simulink model "ASM_Traffic_new"  (R2024a)
settings: Solver=ode1  StartTime=SIM.tstart.v  StopTime=SIM.tend.v  FixedStep=SIM.StepSize.v  RelTol=1e-3
PostLoadFcn:
  | if any(exist('dsrtsu_mdlpostloadfcn', 'file') ~= 0), dsrtsu_mdlpostloadfcn('Execute', bdroot); end
  | try, asm_mdl_postloadfcn(bdroot, 'UpdateModel', 3600); catch, disp(lasterr); end,
InitFcn:
  | , if any(exist('rtifpga_mdlclblib', 'file') ~= 0), rtifpga_mdlclblib('Init', bdroot); end,
  | , if any(exist('dsmpb_private', 'file') ~= 0), dsmpb_private('dsmpb_mdlclblib', 'Init', bdroot); end,
undefined symbols (not defined in the file): _to_, a0b2, ASM_BrakeHydraulics_DemoSystems, ASM_VehicleDynamics_DemoSystems, b98103fe8ad365046cd0, BrakeCircuit, CPT, Crankshaft, DiscIntNeverNeededParam, dsmsi, FinalDriveAssembly, MDL, ModeSignals, Pos_BrakePedal_Maneuver, rad, RefSignals, s_to_rpm, SIM, SoftECU, Suspension, Tire, Transmission
libraries: ASM_Traffic_lib x135, simulink x100, ASM_Utils_lib x77, ASM_VehicleDynamics_lib x70, ASM_Environment_lib x22, dsmpblib x20, dsmsilib x15, MDLD_Utils_lib x10, ASM_BrakeHydraulics_lib x3
(part 60 of 63)

== system ASM_Traffic_new/Environment/Sensors/UserInterface/DISP_Plant/Object_Sensor_3D/Object_Sensor_3D_VisualizationData/Sensor_3_Rear_NearestPoints ==
  Sensor : Inport
  Angle_Hor_Point[deg] : Gain
  Angle_Orientation_Sensor_CoorSys_V[x;y;z][deg] : Gain
  Angle_ScopeZone_Horizontal[deg] : Gain
  Bus Selector : BusSelector  OutputSignals=Parameter.Sensor_Enable[0Off|1On],Parameter.Geometry[],Parameter.Pos_Sensor_Apex_CoorSys_V[x;y;z][m],Parameter.Angle_Orientation_Sensor_CoorSys_V[x;y;z][deg],Parameter.Length_ScopeZone[m],Parameter.Length_ScopeZone_Head[m],Parameter.Angle_ScopeZone_Horizontal[deg],Parameter.Length_BlindZone[m],Parameter.SensorIdx[],SensorOutput.Object_ID[],SensorOutput.Dist_Object[m],SensorOutput.Angle_Hor_Object[deg]
  Dist_Point[m] : Gain
  Geometry[] : Gain
  Length_BlindZone[m] : Gain
  Length_ScopeZone[m] : Gain
  Length_ScopeZone_Head[m] : Gain
  Object_ID_Point[] : Gain
  Pos_Sensor_Apex_CoorSys_V[x;y;z][m] : Gain
  SensorIdx[] : Gain
  Sensor_Enable[0Off|1On] : Gain
  Terminator{9..20} (12 alike) : Terminator
  wires:
  Sensor/1 -> Bus Selector/1
  Length_BlindZone[m]/1 -> Terminator12/1
  Angle_ScopeZone_Horizontal[deg]/1 -> Terminator15/1
  Sensor_Enable[0Off|1On]/1 -> Terminator10/1
  Length_ScopeZone[m]/1 -> Terminator17/1
  Dist_Point[m]/1 -> Terminator9/1
  Angle_Orientation_Sensor_CoorSys_V[x;y;z][deg]/1 -> Terminator18/1
  Angle_Hor_Point[deg]/1 -> Terminator19/1
  SensorIdx[]/1 -> Terminator14/1
  Length_ScopeZone_Head[m]/1 -> Terminator16/1
  Pos_Sensor_Apex_CoorSys_V[x;y;z][m]/1 -> Terminator20/1
  Geometry[]/1 -> Terminator11/1
  Object_ID_Point[]/1 -> Terminator13/1
  Bus Selector/1 -> Sensor_Enable[0Off|1On]/1  "<Sensor_Enable[0Off|1On]>"
  Bus Selector/2 -> Geometry[]/1  "<Geometry[]>"
  Bus Selector/3 -> Pos_Sensor_Apex_CoorSys_V[x;y;z][m]/1  "<Pos_Sensor_Apex_CoorSys_V[x;y;z][m]>"
  Bus Selector/4 -> Angle_Orientation_Sensor_CoorSys_V[x;y;z][deg]/1  "<Angle_Orientation_Sensor_CoorSys_V[x;y;z][deg]>"
  Bus Selector/5 -> Length_ScopeZone[m]/1  "<Length_ScopeZone[m]>"
  Bus Selector/6 -> Length_ScopeZone_Head[m]/1  "<Length_ScopeZone_Head[m]>"
  Bus Selector/7 -> Angle_ScopeZone_Horizontal[deg]/1  "<Angle_ScopeZone_Horizontal[deg]>"
  Bus Selector/8 -> Length_BlindZone[m]/1  "<Length_BlindZone[m]>"
  Bus Selector/9 -> SensorIdx[]/1  "<SensorIdx[]>"
  Bus Selector/11 -> Dist_Point[m]/1  "<Dist_Object[m]>"
  Bus Selector/10 -> Object_ID_Point[]/1  "<Object_ID[]>"
  Bus Selector/12 -> Angle_Hor_Point[deg]/1  "<Angle_Hor_Object[deg]>"

== system ASM_Traffic_new/Environment/Sensors/UserInterface/DISP_Plant/Object_Sensor_3D/Object_Sensor_3D_VisualizationData/Sensor_3_Rear_RadarReflectionPoints ==
  Sensor : Inport
  Angle_Hor_Point[deg] : Gain
  Angle_Orientation_Sensor_CoorSys_V[x;y;z][deg] : Gain
  Angle_ScopeZone_Horizontal[deg] : Gain
  Bus Selector : BusSelector  OutputSignals=Parameter.Sensor_Enable[0Off|1On],Parameter.Geometry[],Parameter.Pos_Sensor_Apex_CoorSys_V[x;y;z][m],Parameter.Angle_Orientation_Sensor_CoorSys_V[x;y;z][deg],Parameter.Length_ScopeZone[m],Parameter.Length_ScopeZone_Head[m],Parameter.Angle_ScopeZone_Horizontal[deg],Parameter.Length_BlindZone[m],Parameter.SensorIdx[],RadarEffects.Object_ID[],RadarEffects.Dist_CoorSys_S[m],RadarEffects.Angle_Hor_CoorSys_S[deg]
  Dist_Point[m] : Gain
  Geometry[] : Gain
  Length_BlindZone[m] : Gain
  Length_ScopeZone[m] : Gain
  Length_ScopeZone_Head[m] : Gain
  Object_ID_Point[] : Gain
  Pos_Sensor_Apex_CoorSys_V[x;y;z][m] : Gain
  SensorIdx[] : Gain
  Sensor_Enable[0Off|1On] : Gain
  Terminator{9..20} (12 alike) : Terminator
  wires:
  Bus Selector/12 -> Angle_Hor_Point[deg]/1  "<Angle_Hor_CoorSys_S[deg]>"
  Bus Selector/10 -> Object_ID_Point[]/1  "<Object_ID[]>"
  Bus Selector/11 -> Dist_Point[m]/1  "<Dist_CoorSys_S[m]>"
  Bus Selector/9 -> SensorIdx[]/1  "<SensorIdx[]>"
  Bus Selector/8 -> Length_BlindZone[m]/1  "<Length_BlindZone[m]>"
  Bus Selector/7 -> Angle_ScopeZone_Horizontal[deg]/1  "<Angle_ScopeZone_Horizontal[deg]>"
  Bus Selector/6 -> Length_ScopeZone_Head[m]/1  "<Length_ScopeZone_Head[m]>"
  Bus Selector/5 -> Length_ScopeZone[m]/1  "<Length_ScopeZone[m]>"
  Bus Selector/4 -> Angle_Orientation_Sensor_CoorSys_V[x;y;z][deg]/1  "<Angle_Orientation_Sensor_CoorSys_V[x;y;z][deg]>"
  Bus Selector/3 -> Pos_Sensor_Apex_CoorSys_V[x;y;z][m]/1  "<Pos_Sensor_Apex_CoorSys_V[x;y;z][m]>"
  Bus Selector/2 -> Geometry[]/1  "<Geometry[]>"
  Bus Selector/1 -> Sensor_Enable[0Off|1On]/1  "<Sensor_Enable[0Off|1On]>"
  Object_ID_Point[]/1 -> Terminator13/1
  Geometry[]/1 -> Terminator11/1
  Pos_Sensor_Apex_CoorSys_V[x;y;z][m]/1 -> Terminator20/1
  Length_ScopeZone_Head[m]/1 -> Terminator16/1
  SensorIdx[]/1 -> Terminator14/1
  Angle_Hor_Point[deg]/1 -> Terminator19/1
  Angle_Orientation_Sensor_CoorSys_V[x;y;z][deg]/1 -> Terminator18/1
  Dist_Point[m]/1 -> Terminator9/1
  Length_ScopeZone[m]/1 -> Terminator17/1
  Sensor_Enable[0Off|1On]/1 -> Terminator10/1
  Angle_ScopeZone_Horizontal[deg]/1 -> Terminator15/1
  Length_BlindZone[m]/1 -> Terminator12/1
  Sensor/1 -> Bus Selector/1

== system ASM_Traffic_new/Environment/Sensors/UserInterface/DISP_Plant/Traffic_Sign_Sensor/GetTrfSgnDataByIndex_1/SwitchObjectData ==
  TrafficBus : Inport
  Switch : Inport  Port=2
  Bus Selector2 : BusSelector  OutputSignals=TrafficSign_Sensor_Dyn.Sensor_Front_1.SensorOutput[].TrafficObject_Type[]
  Bus Selector3 : BusSelector  OutputSignals=TrafficSign_Sensor_Dyn.Sensor_Front_1.SensorOutput[].TrafficObject_ID[]
  Bus Selector4 : BusSelector  OutputSignals=TrafficSign_Sensor_Dyn.Sensor_Front_1.SensorOutput[].Parent_Object_ID[]
  Bus Selector44 : BusSelector  OutputSignals=TrafficSign_Sensor_Dyn.Sensor_Front_1.SensorOutput[].Traffic_Sign_Valid[0|1]
  Selector{,1..3} (4 alike) : Selector  InputPortWidth=MDL.Traffic.Sensors.TrafficSignSensorDyn_Calculation.Const_Sensor_Output_Dimension.v  IndexOptions=Index vector (port)  Indices=[1 3]  OutputSizes=1
  Traffic_Sign_Valid[0|1] : Outport  VectorParamsAs1DForOutWhenUnconnected=off
  TrafficObject_ID[] : Outport  Port=2  VectorParamsAs1DForOutWhenUnconnected=off
  TrafficObject_Type[] : Outport  Port=3  VectorParamsAs1DForOutWhenUnconnected=off
  Parent_Object_ID[] : Outport  Port=4  VectorParamsAs1DForOutWhenUnconnected=off
  wires:
  Selector3/1 -> Parent_Object_ID[]/1
  Bus Selector4/1 -> Selector3/1  "<Parent_Object_ID[]>"
  Selector2/1 -> TrafficObject_Type[]/1
  Switch/1 -> Selector/2, Selector1/2, Selector2/2, Selector3/2
  Selector/1 -> Traffic_Sign_Valid[0|1]/1
  Bus Selector44/1 -> Selector/1  "<Traffic_Sign_Valid[0|1]>"
  Selector1/1 -> TrafficObject_ID[]/1
  Bus Selector3/1 -> Selector1/1  "<TrafficObject_ID[]>"
  TrafficBus/1 -> Bus Selector44/1, Bus Selector3/1, Bus Selector2/1, Bus Selector4/1
  Bus Selector2/1 -> Selector2/1  "<TrafficObject_Type[]>"

== system ASM_Traffic_new/Environment/Sensors/UserInterface/DISP_Plant/Traffic_Sign_Sensor/GetTrfSgnDataByIndex_1/SwitchObjectPosition ==
  TrafficBus : Inport
  Switch : Inport  Port=2
  Bus Selector1 : BusSelector  OutputSignals=TrafficSign_Sensor_Dyn.Sensor_Front_1.SensorOutput[].Pos_CoorSys_S[x;y;z][m]
  Bus Selector2 : BusSelector  OutputSignals=TrafficSign_Sensor_Dyn.Sensor_Front_1.SensorOutput[].Angle_Hor_Rel[deg]
  Bus Selector3 : BusSelector  OutputSignals=TrafficSign_Sensor_Dyn.Sensor_Front_1.SensorOutput[].Angle_CoorSys_E[x;y;z][deg]
  Bus Selector4 : BusSelector  OutputSignals=TrafficSign_Sensor_Dyn.Sensor_Front_1.SensorOutput[].Angle_Ver_Rel[deg]
  Bus Selector44 : BusSelector  OutputSignals=TrafficSign_Sensor_Dyn.Sensor_Front_1.SensorOutput[].Pos_CoorSys_E[x;y;z][m]
  Bus Selector5 : BusSelector  OutputSignals=TrafficSign_Sensor_Dyn.Sensor_Front_1.SensorOutput[].Distance[m]
  Idx_comp : Subsystem
  Idx_comp1 : Subsystem
  Idx_comp2 : Subsystem
  Mux : Mux  Inputs=3
  Mux1 : Mux  Inputs=3
  Mux2 : Mux  Inputs=3
  Selector{1..9} (9 alike) : Selector  InputPortWidth=MDL.Traffic.Sensors.TrafficSignSensorDyn_Calculation.Const_Sensor_Output_Dimension.v*3  IndexOptions=Index vector (port)  Indices=[1 3]  OutputSizes=1
  Selector10 : Selector  InputPortWidth=MDL.Traffic.Sensors.TrafficSignSensorDyn_Calculation.Const_Sensor_Output_Dimension.v  IndexOptions=Index vector (port)  Indices=[1 3]  OutputSizes=1
  Selector11 : Selector  InputPortWidth=MDL.Traffic.Sensors.TrafficSignSensorDyn_Calculation.Const_Sensor_Output_Dimension.v  IndexOptions=Index vector (port)  Indices=[1 3]  OutputSizes=1
  Selector12 : Selector  InputPortWidth=MDL.Traffic.Sensors.TrafficSignSensorDyn_Calculation.Const_Sensor_Output_Dimension.v  IndexOptions=Index vector (port)  Indices=[1 3]  OutputSizes=1
  Pos_CoorSys_E[x;y;z][m] : Outport  VectorParamsAs1DForOutWhenUnconnected=off
  Angle_CoorSys_E[x;y;z][deg] : Outport  Port=2  VectorParamsAs1DForOutWhenUnconnected=off
  Pos_CoorSys_S[x;y;z][m] : Outport  Port=3  VectorParamsAs1DForOutWhenUnconnected=off
  Angle_Hor_Rel[deg] : Outport  Port=4  VectorParamsAs1DForOutWhenUnconnected=off
  Angle_Ver_Rel[deg] : Outport  Port=5  VectorParamsAs1DForOutWhenUnconnected=off
  Distance[m] : Outport  Port=6  VectorParamsAs1DForOutWhenUnconnected=off
  wires:
  Selector12/1 -> Distance[m]/1
  Selector11/1 -> Angle_Ver_Rel[deg]/1
  Selector10/1 -> Angle_Hor_Rel[deg]/1
  Bus Selector5/1 -> Selector12/1  "<Distance[m]>"
  Bus Selector4/1 -> Selector11/1  "<Angle_Ver_Rel[deg]>"
  Bus Selector2/1 -> Selector10/1  "<Angle_Hor_Rel[deg]>"
  Mux2/1 -> Pos_CoorSys_S[x;y;z][m]/1
  Idx_comp2/3(Idx_comp_z) -> Selector9/2
  Idx_comp2/2(Idx_comp_y) -> Selector8/2
  Idx_comp2/1(Idx_comp_x) -> Selector7/2
  Selector9/1 -> Mux2/3
  Selector8/1 -> Mux2/2
  Selector7/1 -> Mux2/1
  Bus Selector1/1 -> Selector7/1, Selector8/1, Selector9/1  "<Pos_CoorSys_S[x;y;z][m]>"
  Mux1/1 -> Angle_CoorSys_E[x;y;z][deg]/1
  Selector3/1 -> Mux1/3
  Selector2/1 -> Mux1/2
  Selector1/1 -> Mux1/1
  Idx_comp1/3(Idx_comp_z) -> Selector3/2
  Idx_comp1/2(Idx_comp_y) -> Selector2/2
  Idx_comp1/1(Idx_comp_x) -> Selector1/2
  Mux/1 -> Pos_CoorSys_E[x;y;z][m]/1
  Selector6/1 -> Mux/3
  Selector5/1 -> Mux/2
  Selector4/1 -> Mux/1
  Idx_comp/3(Idx_comp_z) -> Selector6/2
  Idx_comp/2(Idx_comp_y) -> Selector5/2
  Idx_comp/1(Idx_comp_x) -> Selector4/2
  TrafficBus/1 -> Bus Selector3/1, Bus Selector4/1, Bus Selector5/1, Bus Selector2/1, Bus Selector1/1, Bus Selector44/1
  Bus Selector3/1 -> Selector1/1, Selector2/1, Selector3/1  "<Angle_CoorSys_E[x;y;z][deg]>"
  Bus Selector44/1 -> Selector4/1, Selector5/1, Selector6/1  "<Pos_CoorSys_E[x;y;z][m]>"
  Switch/1 -> Idx_comp/1(Idx), Idx_comp1/1(Idx), Idx_comp2/1(Idx), Selector10/2, Selector11/2, Selector12/2

== system ASM_Traffic_new/Environment/Sensors/UserInterface/DISP_Plant/Traffic_Sign_Sensor/GetTrfSgnDataByIndex_1/SwitchSignProperties ==
  TrafficBus : Inport
  Switch : Inport  Port=2
  Bus Selector1 : BusSelector  OutputSignals=TrafficSign_Sensor_Dyn.Sensor_Front_1.SensorOutput[].Traffic_Sign_Visibility[0_100]
  Bus Selector2 : BusSelector  OutputSignals=TrafficSign_Sensor_Dyn.Sensor_Front_1.SensorOutput[].Traffic_Sign_Value[]
  Bus Selector3 : BusSelector  OutputSignals=TrafficSign_Sensor_Dyn.Sensor_Front_1.SensorOutput[].Traffic_Sign_Subtype[]
  Bus Selector4 : BusSelector  OutputSignals=TrafficSign_Sensor_Dyn.Sensor_Front_1.SensorOutput[].Traffic_Sign_Country[]
  Bus Selector44 : BusSelector  OutputSignals=TrafficSign_Sensor_Dyn.Sensor_Front_1.SensorOutput[].Traffic_Sign_Type[]
  Bus Selector5 : BusSelector  OutputSignals=TrafficSign_Sensor_Dyn.Sensor_Front_1.SensorOutput[].Traffic_Sign_Lanes[]
  Bus Selector6 : BusSelector  OutputSignals=TrafficSign_Sensor_Dyn.Sensor_Front_1.SensorOutput[].Object_State[]
  Bus Selector7 : BusSelector  OutputSignals=TrafficSign_Sensor_Dyn.Sensor_Front_1.SensorOutput[].Object_Stream_ID[]
  Idx_comp : Subsystem
  Mux2 : Mux  Inputs=5
  Selector{,1..3,6,10..11} (7 alike) : Selector  InputPortWidth=MDL.Traffic.Sensors.TrafficSignSensorDyn_Calculation.Const_Sensor_Output_Dimension.v  IndexOptions=Index vector (port)  Indices=[1 3]  OutputSizes=1
  Selector{4..5,7..9} (5 alike) : Selector  InputPortWidth=MDL.Traffic.Sensors.TrafficSignSensorDyn_Calculation.Const_Sensor_Output_Dimension.v*5  IndexOptions=Index vector (port)  Indices=[1 3]  OutputSizes=1
  Traffic_Sign_Type[] : Outport  VectorParamsAs1DForOutWhenUnconnected=off
  Traffic_Sign_Subtype[] : Outport  Port=2  VectorParamsAs1DForOutWhenUnconnected=off
  Traffic_Sign_Value[] : Outport  Port=3  VectorParamsAs1DForOutWhenUnconnected=off
  Traffic_Sign_Country[] : Outport  Port=4  VectorParamsAs1DForOutWhenUnconnected=off
  Traffic_Sign_Visibility[0_100] : Outport  Port=5  VectorParamsAs1DForOutWhenUnconnected=off
  Object_State[] : Outport  Port=6  VectorParamsAs1DForOutWhenUnconnected=off
  Object_Stream_ID[] : Outport  Port=7  VectorParamsAs1DForOutWhenUnconnected=off
  Traffic_Sign_Lanes[] : Outport  Port=8  VectorParamsAs1DForOutWhenUnconnected=off
  wires:
  Bus Selector7/1 -> Selector11/1  "<Object_Stream_ID[]>"
  Selector11/1 -> Object_Stream_ID[]/1
  Bus Selector6/1 -> Selector10/1  "<Object_State[]>"
  Selector10/1 -> Object_State[]/1
  Selector6/1 -> Traffic_Sign_Visibility[0_100]/1
  Selector4/1 -> Mux2/4
  Idx_comp/4(Idx_comp_4) -> Selector4/2
  Idx_comp/5(Idx_comp_5) -> Selector5/2
  Selector5/1 -> Mux2/5
  Mux2/1 -> Traffic_Sign_Lanes[]/1
  Idx_comp/3(Idx_comp_3) -> Selector9/2
  Idx_comp/2(Idx_comp_2) -> Selector8/2
  Idx_comp/1(Idx_comp_1) -> Selector7/2
  Selector9/1 -> Mux2/3
  Selector8/1 -> Mux2/2
  Selector7/1 -> Mux2/1
  Bus Selector5/1 -> Selector7/1, Selector8/1, Selector9/1, Selector5/1, Selector4/1  "<Traffic_Sign_Lanes[]>"
  Bus Selector1/1 -> Selector6/1  "<Traffic_Sign_Visibility[0_100]>"
  Bus Selector2/1 -> Selector2/1  "<Traffic_Sign_Value[]>"
  TrafficBus/1 -> Bus Selector4/1, Bus Selector1/1, Bus Selector7/1, Bus Selector5/1, Bus Selector6/1, Bus Selector2/1, Bus Selector3/1, Bus Selector44/1
  Bus Selector3/1 -> Selector1/1  "<Traffic_Sign_Subtype[]>"
  Selector1/1 -> Traffic_Sign_Subtype[]/1
  Bus Selector44/1 -> Selector/1  "<Traffic_Sign_Type[]>"
  Selector/1 -> Traffic_Sign_Type[]/1
  Switch/1 -> Selector3/2, Selector10/2, Idx_comp/1(Idx), Selector11/2, Selector6/2, Selector2/2, Selector1/2, Selector/2
  Selector2/1 -> Traffic_Sign_Value[]/1
  Bus Selector4/1 -> Selector3/1  "<Traffic_Sign_Country[]>"
  Selector3/1 -> Traffic_Sign_Country[]/1

== system ASM_Traffic_new/Environment/Traffic/UserInterface/DISP_Plant/Fellow_Movement/GetFellowDataByIndex_1/SwitchFellowMovementData ==
  TrafficBus : Inport
  Switch : Inport  Port=2
  Bus Selector2 : BusSelector  OutputSignals=Traffic_Signals_toEnvironment.Flag_FellowUsed[0|1]
  Bus Selector3 : BusSelector  OutputSignals=FellowSignalLabels.s_Fellows[m]
  Bus Selector4 : BusSelector  OutputSignals=FellowSignalLabels.d_Total_Fellows[m]
  Bus Selector5 : BusSelector  OutputSignals=FellowSignalLabels.v_Fellows[km|h]
  Flag_Fellow_Used[0|1] : Subsystem
      mask Display: disp('')
  Selector{,1..3} (4 alike) : Selector  InputPortWidth=MDL.Traffic.MaxNumFellows.v  IndexOptions=Index vector (port)  Indices=[1 3]  OutputSizes=1
  d_Total_Fellow[m] : Subsystem
      mask Display: disp('')
  s_Fellow[m] : Subsystem
      mask Display: disp('')
  v_Fellow[km|h] : Subsystem
      mask Display: disp('')
  "Flag_Fellow_Used[0|1] " : Outport  VectorParamsAs1DForOutWhenUnconnected=off
  "s_Fellow[m] " : Outport  Port=2  VectorParamsAs1DForOutWhenUnconnected=off
  "d_Total_Fellow[m] " : Outport  Port=3  VectorParamsAs1DForOutWhenUnconnected=off
  "v_Fellow[km|h] " : Outport  Port=4  VectorParamsAs1DForOutWhenUnconnected=off
  wires:
  TrafficBus/1 -> Bus Selector2/1, Bus Selector3/1, Bus Selector4/1, Bus Selector5/1
  Selector3/1 -> v_Fellow[km|h]/1(In1)
  Bus Selector5/1 -> Selector3/1  "<v_Fellows[km|h]>"
  Selector2/1 -> d_Total_Fellow[m]/1(In1)
  Bus Selector4/1 -> Selector2/1  "<d_Total_Fellows[m]>"
  Selector1/1 -> s_Fellow[m]/1(In1)
  Bus Selector3/1 -> Selector1/1  "<s_Fellows[m]>"
  Selector/1 -> Flag_Fellow_Used[0|1]/1(In1)
  Bus Selector2/1 -> Selector/1  "<Flag_FellowUsed[0|1]>"
  Switch/1 -> Selector/2, Selector1/2, Selector2/2, Selector3/2
  v_Fellow[km|h]/1(Out1) -> "v_Fellow[km|h] "/1  "v_Fellow[km|h]"
  d_Total_Fellow[m]/1(Out1) -> "d_Total_Fellow[m] "/1  "d_Total_Fellow[m]"
  s_Fellow[m]/1(Out1) -> "s_Fellow[m] "/1  "s_Fellow[m]"
  Flag_Fellow_Used[0|1]/1(Out1) -> "Flag_Fellow_Used[0|1] "/1  "Flag_Fellow_Used[0|1]"

== system ASM_Traffic_new/Environment/Traffic/UserInterface/DISP_Plant/Fellow_Movement/GetFellowDataByIndex_1/SwitchInfoData ==
  TrafficBus : Inport
  Switch : Inport  Port=2
  Bus Selector1 : BusSelector  OutputSignals=Traffic_Signals_toEnvironment.Info.CurrentSegment_Fellows[]
  Bus Selector2 : BusSelector  OutputSignals=Traffic_Signals_toEnvironment.Info.t_local_Fellows[s]
  Bus Selector44 : BusSelector  OutputSignals=Traffic_Signals_toEnvironment.Info.CurrentSequence_Fellows[]
  Selector : Selector  InputPortWidth=MDL.Traffic.MaxNumFellows.v  IndexOptions=Index vector (port)  Indices=[1 3]  OutputSizes=1
  Selector1 : Selector  InputPortWidth=MDL.Traffic.MaxNumFellows.v  IndexOptions=Index vector (port)  Indices=[1 3]  OutputSizes=1
  Selector2 : Selector  InputPortWidth=MDL.Traffic.MaxNumFellows.v  IndexOptions=Index vector (port)  Indices=[1 3]  OutputSizes=1
  CurrentSequence[] : Outport  VectorParamsAs1DForOutWhenUnconnected=off
  CurrentSegment[] : Outport  Port=2  VectorParamsAs1DForOutWhenUnconnected=off
  t_local[s] : Outport  Port=3  VectorParamsAs1DForOutWhenUnconnected=off
  wires:
  Selector2/1 -> t_local[s]/1
  Switch/1 -> Selector/2, Selector1/2, Selector2/2
  Selector/1 -> CurrentSequence[]/1
  Bus Selector44/1 -> Selector/1  "<CurrentSequence_Fellows[]>"
  Selector1/1 -> CurrentSegment[]/1
  Bus Selector1/1 -> Selector1/1  "<CurrentSegment_Fellows[]>"
  TrafficBus/1 -> Bus Selector44/1, Bus Selector1/1, Bus Selector2/1
  Bus Selector2/1 -> Selector2/1  "<t_local_Fellows[s]>"

== system ASM_Traffic_new/Environment/Traffic/UserInterface/DISP_Plant/Fellow_Movement/GetFellowDataByIndex_2/SwitchFellowMovementData ==
  TrafficBus : Inport
  Switch : Inport  Port=2
  Bus Selector2 : BusSelector  OutputSignals=Traffic_Signals_toEnvironment.Flag_FellowUsed[0|1]
  Bus Selector3 : BusSelector  OutputSignals=FellowSignalLabels.s_Fellows[m]
  Bus Selector4 : BusSelector  OutputSignals=FellowSignalLabels.d_Total_Fellows[m]
  Bus Selector5 : BusSelector  OutputSignals=FellowSignalLabels.v_Fellows[km|h]
  Flag_Fellow_Used[0|1] : Subsystem
      mask Display: disp('')
  Selector{,1..3} (4 alike) : Selector  InputPortWidth=MDL.Traffic.MaxNumFellows.v  IndexOptions=Index vector (port)  Indices=[1 3]  OutputSizes=1
  d_Total_Fellow[m] : Subsystem
      mask Display: disp('')
  s_Fellow[m] : Subsystem
      mask Display: disp('')
  v_Fellow[km|h] : Subsystem
      mask Display: disp('')
  "Flag_Fellow_Used[0|1] " : Outport  VectorParamsAs1DForOutWhenUnconnected=off
  "s_Fellow[m] " : Outport  Port=2  VectorParamsAs1DForOutWhenUnconnected=off
  "d_Total_Fellow[m] " : Outport  Port=3  VectorParamsAs1DForOutWhenUnconnected=off
  "v_Fellow[km|h] " : Outport  Port=4  VectorParamsAs1DForOutWhenUnconnected=off
  wires:
  TrafficBus/1 -> Bus Selector2/1, Bus Selector3/1, Bus Selector4/1, Bus Selector5/1
  Selector3/1 -> v_Fellow[km|h]/1(In1)
  Bus Selector5/1 -> Selector3/1  "<v_Fellows[km|h]>"
  Selector2/1 -> d_Total_Fellow[m]/1(In1)
  Bus Selector4/1 -> Selector2/1  "<d_Total_Fellows[m]>"
  Selector1/1 -> s_Fellow[m]/1(In1)
  Bus Selector3/1 -> Selector1/1  "<s_Fellows[m]>"
  Selector/1 -> Flag_Fellow_Used[0|1]/1(In1)
  Bus Selector2/1 -> Selector/1  "<Flag_FellowUsed[0|1]>"
  Switch/1 -> Selector/2, Selector1/2, Selector2/2, Selector3/2
  v_Fellow[km|h]/1(Out1) -> "v_Fellow[km|h] "/1  "v_Fellow[km|h]"
  d_Total_Fellow[m]/1(Out1) -> "d_Total_Fellow[m] "/1  "d_Total_Fellow[m]"
  s_Fellow[m]/1(Out1) -> "s_Fellow[m] "/1  "s_Fellow[m]"
  Flag_Fellow_Used[0|1]/1(Out1) -> "Flag_Fellow_Used[0|1] "/1  "Flag_Fellow_Used[0|1]"

== system ASM_Traffic_new/Environment/Traffic/UserInterface/DISP_Plant/Fellow_Movement/GetFellowDataByIndex_2/SwitchInfoData ==
  TrafficBus : Inport
  Switch : Inport  Port=2
  Bus Selector1 : BusSelector  OutputSignals=Traffic_Signals_toEnvironment.Info.CurrentSegment_Fellows[]
  Bus Selector2 : BusSelector  OutputSignals=Traffic_Signals_toEnvironment.Info.t_local_Fellows[s]
  Bus Selector44 : BusSelector  OutputSignals=Traffic_Signals_toEnvironment.Info.CurrentSequence_Fellows[]
  Selector : Selector  InputPortWidth=MDL.Traffic.MaxNumFellows.v  IndexOptions=Index vector (port)  Indices=[1 3]  OutputSizes=1
  Selector1 : Selector  InputPortWidth=MDL.Traffic.MaxNumFellows.v  IndexOptions=Index vector (port)  Indices=[1 3]  OutputSizes=1
  Selector2 : Selector  InputPortWidth=MDL.Traffic.MaxNumFellows.v  IndexOptions=Index vector (port)  Indices=[1 3]  OutputSizes=1
  CurrentSequence[] : Outport  VectorParamsAs1DForOutWhenUnconnected=off
  CurrentSegment[] : Outport  Port=2  VectorParamsAs1DForOutWhenUnconnected=off
  t_local[s] : Outport  Port=3  VectorParamsAs1DForOutWhenUnconnected=off
  wires:
  Selector2/1 -> t_local[s]/1
  Switch/1 -> Selector/2, Selector1/2, Selector2/2
  Selector/1 -> CurrentSequence[]/1
  Bus Selector44/1 -> Selector/1  "<CurrentSequence_Fellows[]>"
  Selector1/1 -> CurrentSegment[]/1
  Bus Selector1/1 -> Selector1/1  "<CurrentSegment_Fellows[]>"
  TrafficBus/1 -> Bus Selector44/1, Bus Selector1/1, Bus Selector2/1
  Bus Selector2/1 -> Selector2/1  "<t_local_Fellows[s]>"

== system ASM_Traffic_new/Environment/Traffic/UserInterface/DISP_Plant/Fellow_Movement/GetFellowDataByIndex_3/SwitchFellowMovementData ==
  TrafficBus : Inport
  Switch : Inport  Port=2
  Bus Selector2 : BusSelector  OutputSignals=Traffic_Signals_toEnvironment.Flag_FellowUsed[0|1]
  Bus Selector3 : BusSelector  OutputSignals=FellowSignalLabels.s_Fellows[m]
  Bus Selector4 : BusSelector  OutputSignals=FellowSignalLabels.d_Total_Fellows[m]
  Bus Selector5 : BusSelector  OutputSignals=FellowSignalLabels.v_Fellows[km|h]
  Flag_Fellow_Used[0|1] : Subsystem
      mask Display: disp('')
  Selector{,1..3} (4 alike) : Selector  InputPortWidth=MDL.Traffic.MaxNumFellows.v  IndexOptions=Index vector (port)  Indices=[1 3]  OutputSizes=1
  d_Total_Fellow[m] : Subsystem
      mask Display: disp('')
  s_Fellow[m] : Subsystem
      mask Display: disp('')
  v_Fellow[km|h] : Subsystem
      mask Display: disp('')
  "Flag_Fellow_Used[0|1] " : Outport  VectorParamsAs1DForOutWhenUnconnected=off
  "s_Fellow[m] " : Outport  Port=2  VectorParamsAs1DForOutWhenUnconnected=off
  "d_Total_Fellow[m] " : Outport  Port=3  VectorParamsAs1DForOutWhenUnconnected=off
  "v_Fellow[km|h] " : Outport  Port=4  VectorParamsAs1DForOutWhenUnconnected=off
  wires:
  TrafficBus/1 -> Bus Selector2/1, Bus Selector3/1, Bus Selector4/1, Bus Selector5/1
  Selector3/1 -> v_Fellow[km|h]/1(In1)
  Bus Selector5/1 -> Selector3/1  "<v_Fellows[km|h]>"
  Selector2/1 -> d_Total_Fellow[m]/1(In1)
  Bus Selector4/1 -> Selector2/1  "<d_Total_Fellows[m]>"
  Selector1/1 -> s_Fellow[m]/1(In1)
  Bus Selector3/1 -> Selector1/1  "<s_Fellows[m]>"
  Selector/1 -> Flag_Fellow_Used[0|1]/1(In1)
  Bus Selector2/1 -> Selector/1  "<Flag_FellowUsed[0|1]>"
  Switch/1 -> Selector/2, Selector1/2, Selector2/2, Selector3/2
  v_Fellow[km|h]/1(Out1) -> "v_Fellow[km|h] "/1  "v_Fellow[km|h]"
  d_Total_Fellow[m]/1(Out1) -> "d_Total_Fellow[m] "/1  "d_Total_Fellow[m]"
  s_Fellow[m]/1(Out1) -> "s_Fellow[m] "/1  "s_Fellow[m]"
  Flag_Fellow_Used[0|1]/1(Out1) -> "Flag_Fellow_Used[0|1] "/1  "Flag_Fellow_Used[0|1]"

== system ASM_Traffic_new/Environment/Traffic/UserInterface/DISP_Plant/Fellow_Movement/GetFellowDataByIndex_3/SwitchInfoData ==
  TrafficBus : Inport
  Switch : Inport  Port=2
  Bus Selector1 : BusSelector  OutputSignals=Traffic_Signals_toEnvironment.Info.CurrentSegment_Fellows[]
  Bus Selector2 : BusSelector  OutputSignals=Traffic_Signals_toEnvironment.Info.t_local_Fellows[s]
  Bus Selector44 : BusSelector  OutputSignals=Traffic_Signals_toEnvironment.Info.CurrentSequence_Fellows[]
  Selector : Selector  InputPortWidth=MDL.Traffic.MaxNumFellows.v  IndexOptions=Index vector (port)  Indices=[1 3]  OutputSizes=1
  Selector1 : Selector  InputPortWidth=MDL.Traffic.MaxNumFellows.v  IndexOptions=Index vector (port)  Indices=[1 3]  OutputSizes=1
  Selector2 : Selector  InputPortWidth=MDL.Traffic.MaxNumFellows.v  IndexOptions=Index vector (port)  Indices=[1 3]  OutputSizes=1
  CurrentSequence[] : Outport  VectorParamsAs1DForOutWhenUnconnected=off
  CurrentSegment[] : Outport  Port=2  VectorParamsAs1DForOutWhenUnconnected=off
  t_local[s] : Outport  Port=3  VectorParamsAs1DForOutWhenUnconnected=off
  wires:
  Selector2/1 -> t_local[s]/1
  Switch/1 -> Selector/2, Selector1/2, Selector2/2
  Selector/1 -> CurrentSequence[]/1
  Bus Selector44/1 -> Selector/1  "<CurrentSequence_Fellows[]>"
  Selector1/1 -> CurrentSegment[]/1
  Bus Selector1/1 -> Selector1/1  "<CurrentSegment_Fellows[]>"
  TrafficBus/1 -> Bus Selector44/1, Bus Selector1/1, Bus Selector2/1
  Bus Selector2/1 -> Selector2/1  "<t_local_Fellows[s]>"

== system ASM_Traffic_new/VehicleDynamics/Plant/VehicleDynamics/VehicleMovement/ASMSignalCollector/Vehicle_Movement_Info_Car/Accelerations ==
  ASMBUS_VehicleDynamics_MassForcesAndTorques : Inport
  ASMBUS_VehicleDynamics_VehicleMass : Inport  Port=2
  ASMBUS_VehicleDynamics_Suspension : Inport  Port=3
  ASMBUS_VehicleDynamics_Steering : Inport  Port=4
  a_Gravity_CoorSys_V[x;y;z][m|s2] : Inport  Port=5
  v_Vehicle_dt[x;y;z][m|s2] : Inport  Port=6
  w_Vehicle_dt[x;y;z][rad|s2] : Inport  Port=7
  q_Wheel_dt2[q1_Front;q2_Front;q1_Rear;q2_Rear][] : Inport  Port=8
  AbsoluteAcceleration_CoG : Subsystem
  AbsoluteAcceleration_FL : Subsystem
  AbsoluteAcceleration_FR : Subsystem
  AbsoluteAcceleration_RL : Subsystem
  AbsoluteAcceleration_RR : Subsystem
  Bus Selector1 : BusSelector  OutputSignals=SuspensionFront.RelativePositionFront.Pos_Wheel[FL;FR][x;y;z][m].Pos_FL_Wheel[x;y;z][m],SuspensionFront.RelativePositionFront.Pos_Wheel[FL;FR][x;y;z][m].Pos_FR_Wheel[x;y;z][m],SuspensionRear.RelativePositionRear.Pos_Wheel[RL;RR][x;y;z][m].Pos_RL_Wheel[x;y;z][m],SuspensionRear.RelativePositionRear.Pos_Wheel[RL;RR][x;y;z][m].Pos_RR_Wheel[x;y;z][m]
  Bus Selector4 : BusSelector  OutputSignals=PosVec_CoG_TotalVehicle[x;y;z][m]
  Bus Selector5 : BusSelector  OutputSignals=ResidualAccelerations.a_Vehicle_CoG_Residual[x;y;z][m|s2],ResidualAccelerations.a_FL_Residual[x;y;z][m|s2],ResidualAccelerations.a_FR_Residual[x;y;z][m|s2],ResidualAccelerations.a_RL_Residual[x;y;z][m|s2],ResidualAccelerations.a_RR_Residual[x;y;z][m|s2]
  Bus Selector6 : BusSelector  OutputSignals=Displ_SteeringRod_dt2[m|s2]
  BusCreator : BusCreator  Inputs=3
  BusCreator1 : BusCreator  Inputs=3
  BusCreator2 : BusCreator  Inputs=1
  BusCreator3 : BusCreator  Inputs=2
  BusCreator4 : BusCreator  Inputs=4
  BusCreator6 : BusCreator  Inputs=2
  BusCreator7 : BusCreator  Inputs=2
  BusCreator8 : BusCreator  Inputs=1
  Constant : Constant  Value=[0 0 0]
  Demux : Demux  Outputs=3
      settings: DisplayOption=none
  Demux1 : Demux  Outputs=3
      settings: DisplayOption=none
  RelativeAcceleration : Subsystem
  Sum2 : Sum  Inputs=-+  SaturateOnIntegerOverflow=on
  Accelerations : Outport  VectorParamsAs1DForOutWhenUnconnected=off
  wires:
  BusCreator3/1 -> Accelerations/1  "Accelerations"
  BusCreator6/1 -> BusCreator3/1  "VehicleCoG"
  BusCreator8/1 -> BusCreator6/2  "Angular"
  BusCreator7/1 -> BusCreator6/1  "Linear"
  BusCreator2/1 -> BusCreator3/2  "Wheels"
  BusCreator4/1 -> BusCreator2/1  "Linear"
  AbsoluteAcceleration_FL/1(a_i[m|s2]) -> BusCreator4/1  "a_FL_Wheel[x;y;z][m|s2]"
  AbsoluteAcceleration_FR/1(a_i[m|s2]) -> BusCreator4/2  "a_FR_Wheel[x;y;z][m|s2]"
  AbsoluteAcceleration_RL/1(a_i[m|s2]) -> BusCreator4/3  "a_RL_Wheel[x;y;z][m|s2]"
  AbsoluteAcceleration_RR/1(a_i[m|s2]) -> BusCreator4/4  "a_RR_Wheel[x;y;z][m|s2]"
  ASMBUS_VehicleDynamics_Suspension/1 -> Bus Selector1/1, RelativeAcceleration/2(ASMBUS_VehicleDynamics_Suspension)
  Bus Selector1/1 -> AbsoluteAcceleration_FL/3(Pos_i[x;y;z][m])  "<Pos_FL_Wheel[x;y;z][m]>"
  v_Vehicle_dt[x;y;z][m|s2]/1 -> AbsoluteAcceleration_RR/1(v_Vehicle_dt[x;y;z][m|s2]), AbsoluteAcceleration_RL/1(v_Vehicle_dt[x;y;z][m|s2]), AbsoluteAcceleration_FR/1(v_Vehicle_dt[x;y;z][m|s2]), AbsoluteAcceleration_FL/1(v_Vehicle_dt[x;y;z][m|s2]), AbsoluteAcceleration_CoG/1(v_Vehicle_dt[x;y;z][m|s2])
  ASMBUS_VehicleDynamics_VehicleMass/1 -> Bus Selector4/1
  Bus Selector4/1 -> AbsoluteAcceleration_CoG/3(Pos_i[x;y;z][m])  "<PosVec_CoG_TotalVehicle[x;y;z][m]>"
  Bus Selector5/1 -> AbsoluteAcceleration_CoG/4(a_i_Residual[x;y;z][m|s2])  "<a_Vehicle_CoG_Residual[x;y;z][m|s2]>"
  ASMBUS_VehicleDynamics_MassForcesAndTorques/1 -> Bus Selector5/1
  Constant/1 -> AbsoluteAcceleration_CoG/5(Pos_i_dt2[x;y;z][m|s2])
  Bus Selector1/2 -> AbsoluteAcceleration_FR/3(Pos_i[x;y;z][m])  "<Pos_FR_Wheel[x;y;z][m]>"
  Bus Selector1/3 -> AbsoluteAcceleration_RL/3(Pos_i[x;y;z][m])  "<Pos_RL_Wheel[x;y;z][m]>"
  Bus Selector1/4 -> AbsoluteAcceleration_RR/3(Pos_i[x;y;z][m])  "<Pos_RR_Wheel[x;y;z][m]>"
  Bus Selector5/2 -> AbsoluteAcceleration_FL/4(a_i_Residual[x;y;z][m|s2])  "<a_FL_Residual[x;y;z][m|s2]>"
  Bus Selector5/3 -> AbsoluteAcceleration_FR/4(a_i_Residual[x;y;z][m|s2])  "<a_FR_Residual[x;y;z][m|s2]>"
  Bus Selector5/4 -> AbsoluteAcceleration_RL/4(a_i_Residual[x;y;z][m|s2])  "<a_RL_Residual[x;y;z][m|s2]>"
  Bus Selector5/5 -> AbsoluteAcceleration_RR/4(a_i_Residual[x;y;z][m|s2])  "<a_RR_Residual[x;y;z][m|s2]>"
  ASMBUS_VehicleDynamics_Steering/1 -> Bus Selector6/1
  Bus Selector6/1 -> RelativeAcceleration/3(Displ_SteeringRod_dt2[m|s2])  "<Displ_SteeringRod_dt2[m|s2]>"
  RelativeAcceleration/1(Pos_FL_dt2[x;y;z][m|s2]) -> AbsoluteAcceleration_FL/5(Pos_i_dt2[x;y;z][m|s2])
  RelativeAcceleration/2(Pos_FR_dt2[x;y;z][m|s2]) -> AbsoluteAcceleration_FR/5(Pos_i_dt2[x;y;z][m|s2])
  RelativeAcceleration/3(Pos_RL_dt2[x;y;z][m|s2]) -> AbsoluteAcceleration_RL/5(Pos_i_dt2[x;y;z][m|s2])
  RelativeAcceleration/4(Pos_RR_dt2[x;y;z][m|s2]) -> AbsoluteAcceleration_RR/5(Pos_i_dt2[x;y;z][m|s2])
  q_Wheel_dt2[q1_Front;q2_Front;q1_Rear;q2_Rear][]/1 -> RelativeAcceleration/1(q_Wheel_dt2[q1_Front;q2_Front;q1_Rear;q2_Rear][])
  BusCreator/1 -> BusCreator7/1  "a_Vehicle_CoG[x;y;z][m|s2]"
  Demux/3 -> BusCreator/3  "a_z_Vehicle_CoG[m|s2]"
  Demux/2 -> BusCreator/2  "a_y_Vehicle_CoG[m|s2]"
  Demux/1 -> BusCreator/1  "a_x_Vehicle_CoG[m|s2]"
  AbsoluteAcceleration_CoG/1(a_i[m|s2]) -> Demux/1, Sum2/2
  a_Gravity_CoorSys_V[x;y;z][m|s2]/1 -> Sum2/1
  Sum2/1 -> BusCreator7/2  "a_Vehicle_CoG_withG[x;y;z][m|s2]"
  w_Vehicle_dt[x;y;z][rad|s2]/1 -> Demux1/1, AbsoluteAcceleration_CoG/2(w_Vehicle_dt[x;y;z][rad|s2]), AbsoluteAcceleration_FL/2(w_Vehicle_dt[x;y;z][rad|s2]), AbsoluteAcceleration_FR/2(w_Vehicle_dt[x;y;z][rad|s2]), AbsoluteAcceleration_RR/2(w_Vehicle_dt[x;y;z][rad|s2]), AbsoluteAcceleration_RL/2(w_Vehicle_dt[x;y;z][rad|s2])
  Demux1/1 -> BusCreator1/1  "w_x_Vehicle_CoG_dt[rad|s2]"
  Demux1/2 -> BusCreator1/2  "w_y_Vehicle_CoG_dt[rad|s2]"
  Demux1/3 -> BusCreator1/3  "w_z_Vehicle_CoG_dt[rad|s2]"
  BusCreator1/1 -> BusCreator8/1  "w_Vehicle_CoG_dt[x;y;z][rad|s2]"

== system ASM_Traffic_new/VehicleDynamics/Plant/VehicleDynamics/VehicleMovement/ASMSignalCollector/Vehicle_Movement_Info_Car/CoordinateTransformation ==
  a_Gravity_CoorSys_V[x;y;z][m|s2] : Inport
  BusCreator1 : BusCreator  Inputs=1
  CoordinateTransformation : Outport  VectorParamsAs1DForOutWhenUnconnected=off
  wires:
  BusCreator1/1 -> CoordinateTransformation/1  "GravityAcceleration"
  a_Gravity_CoorSys_V[x;y;z][m|s2]/1 -> BusCreator1/1

== system ASM_Traffic_new/VehicleDynamics/Plant/VehicleDynamics/VehicleMovement/ASMSignalCollector/Vehicle_Movement_Info_Car/Positions ==
  Velocities : Inport
  Reset[] : Inport  Port=2
  Pos_Vehicle_CoorSys_E[x;y;z][m] : Inport  Port=3
  Angle_V[Alpha;Beta;Gamma][deg] : Inport  Port=4
  Pos_FL_Wheels_CoorSys_E[x;y;z][m] : Inport  Port=5
  Pos_FR_Wheels_CoorSys_E[x;y;z][m] : Inport  Port=6
  Pos_RL_Wheels_CoorSys_E[x;y;z][m] : Inport  Port=7
  Pos_RR_Wheels_CoorSys_E[x;y;z][m] : Inport  Port=8
  RotationMatrix_V_to_E[3x3] : Inport  Port=9
  RotationMatrix_V_to_E_T[3x3] : Inport  Port=10
  Bus Selector3 : BusSelector  OutputSignals=Vehicle.Linear.v_Total_Vehicle[km|h]
  BusCreator1 : BusCreator  Inputs=1
  BusCreator2 : BusCreator  Inputs=2
  BusCreator3 : BusCreator  Inputs=2
  BusCreator4 : BusCreator  Inputs=3
  BusCreator5 : BusCreator  Inputs=6
  BusCreator6 : BusCreator  Inputs=4
  Discrete-Time Integrator : DiscreteIntegrator  ExternalReset=level  SampleTime=StepSize.v  ICPrevOutput=DiscIntNeverNeededParam  ICPrevScaledInput=DiscIntNeverNeededParam
  UnitConversation : ASM_Utils_lib/UnitConversion/UnitConversion  Selection=km/h_to_m/s
  VectorLabel : Subsystem
  VectorLabel2 : Subsystem
  "[3x3]to[1x9]" : Reshape  OutputDimensionality=Customize  OutputDimensions=[1,9]
  "[3x3]to[1x9]2" : Reshape  OutputDimensionality=Customize  OutputDimensions=[1,9]
  Positions : Outport  VectorParamsAs1DForOutWhenUnconnected=off
  wires:
  UnitConversation/1 -> Discrete-Time Integrator/1
  Bus Selector3/1 -> UnitConversation/1  "<v_Total_Vehicle[km|h]>"
  BusCreator3/1 -> Positions/1  "Positions"
  BusCreator2/1 -> BusCreator3/1  "Vehicle"
  BusCreator4/1 -> BusCreator2/1  "Linear"
  BusCreator1/1 -> BusCreator3/2  "Wheels"
  Pos_FL_Wheels_CoorSys_E[x;y;z][m]/1 -> BusCreator6/1
  Pos_FR_Wheels_CoorSys_E[x;y;z][m]/1 -> BusCreator6/2
  BusCreator6/1 -> BusCreator1/1  "Linear"
  Pos_RL_Wheels_CoorSys_E[x;y;z][m]/1 -> BusCreator6/3
  Pos_RR_Wheels_CoorSys_E[x;y;z][m]/1 -> BusCreator6/4
  Velocities/1 -> Bus Selector3/1
  Reset[]/1 -> Discrete-Time Integrator/2
  Discrete-Time Integrator/1 -> BusCreator4/3  "s_Vehicle[m]"
  Angle_V[Alpha;Beta;Gamma][deg]/1 -> BusCreator5/2, VectorLabel2/1(in)
  BusCreator5/1 -> BusCreator2/2  "Angular"
  RotationMatrix_V_to_E[3x3]/1 -> "[3x3]to[1x9]"/1, BusCreator5/3
  "[3x3]to[1x9]"/1 -> BusCreator5/4  "RotationMatrix_V_to_E[1x9]"
  RotationMatrix_V_to_E_T[3x3]/1 -> "[3x3]to[1x9]2"/1, BusCreator5/5
  "[3x3]to[1x9]2"/1 -> BusCreator5/6  "RotationMatrix_V_to_E_T[1x9]"
  Pos_Vehicle_CoorSys_E[x;y;z][m]/1 -> VectorLabel/1(in), BusCreator4/2  "Pos_Vehicle_CoorSys_E[m]"
  VectorLabel/1(out) -> BusCreator4/1  "Pos_Vehicle_CoorSys_E[x;y;z][m]"
  VectorLabel2/1(out) -> BusCreator5/1

== system ASM_Traffic_new/VehicleDynamics/Plant/VehicleDynamics/VehicleMovement/ASMSignalCollector/Vehicle_Movement_Info_Car/VehicleEquationOfMotion ==
  GeneralizedForcesAndTorques : Inport
  GeneralizedVelocitiesDerivative : Inport  Port=2
  BusCreator1 : BusCreator  Inputs=2
  VehicleEquationOfMotion : Outport  VectorParamsAs1DForOutWhenUnconnected=off
  wires:
  GeneralizedForcesAndTorques/1 -> BusCreator1/1
  BusCreator1/1 -> VehicleEquationOfMotion/1  "VehicleEquationOfMotion"
  GeneralizedVelocitiesDerivative/1 -> BusCreator1/2

== system ASM_Traffic_new/VehicleDynamics/Plant/VehicleDynamics/VehicleMovement/ASMSignalCollector/Vehicle_Movement_Info_Car/Velocities ==
  CoGAndWheelVelocities : Inport
  v_Vehicle[x;y;z][m|s] : Inport  Port=2
  w_Vehicle[x;y;z][rad|s] : Inport  Port=3
  q_Wheel_dt[q1_Front;q2_Front;q1_Rear;q2_Rear][] : Inport  Port=4
  Bus Creator : BusCreator  Inputs=3
  Bus Selector : BusSelector  OutputSignals=v_Abs_Vehicle_CoG[x;y;z][km|h],w_CoG_VehicleBody[x;y;z][rad|s],WheelBodyVelocity,WheelBodyAngularVelocity,WheelAngularVelocity
  BusCreator1 : BusCreator  Inputs=2
  BusCreator2 : BusCreator  Inputs=2
  BusCreator4 : BusCreator  Inputs=3
  BusCreator5 : BusCreator  Inputs=1
  BusCreator6 : BusCreator  Inputs=1
  BusCreator7 : BusCreator  Inputs=2
  BusCreator8 : BusCreator  Inputs=3
  Selector : Selector  InputPortWidth=3  IndexOptions=Index vector (dialog)  Indices=[1 2]  OutputSizes=1
      settings: AttributesFormatString=Elements: %<Elements>
  VectorLabel : Subsystem
  VectorLabel3 : Subsystem
  VectorLabel4 : Subsystem
  "[m|s]_to_[km|h]" : Gain  Gain=3.6
  "[rad]_to_[deg]" : Gain  Gain=180/pi
  "[rad]_to_[deg]1" : Gain  Gain=180/pi
  v_Vehicle_and_AngleSideSlip : Subsystem
  Velocities : Outport  VectorParamsAs1DForOutWhenUnconnected=off
  wires:
  VectorLabel4/1(out) -> BusCreator8/3
  q_Wheel_dt[q1_Front;q2_Front;q1_Rear;q2_Rear][]/1 -> VectorLabel4/1(in)
  "[rad]_to_[deg]1"/1 -> BusCreator8/2  "w_Vehicle[x;y;z][deg|s]"
  "[rad]_to_[deg]"/1 -> VectorLabel3/1(in)
  w_Vehicle[x;y;z][rad|s]/1 -> "[rad]_to_[deg]1"/1
  BusCreator8/1 -> Bus Creator/3  "Generalized"
  v_Vehicle[x;y;z][m|s]/1 -> "[m|s]_to_[km|h]"/1
  "[m|s]_to_[km|h]"/1 -> BusCreator8/1  "v_Vehicle[x;y;z][km|h]"
  CoGAndWheelVelocities/1 -> Bus Selector/1
  BusCreator2/1 -> Bus Creator/1  "Vehicle"
  BusCreator4/1 -> BusCreator2/1  "Linear"
  BusCreator5/1 -> BusCreator2/2  "Angular"
  VectorLabel3/1(out) -> BusCreator5/1
  Bus Creator/1 -> Velocities/1  "Velocities"
  BusCreator1/1 -> Bus Creator/2  "Wheels"
  BusCreator7/1 -> BusCreator1/2  "Angular"
  Bus Selector/1 -> VectorLabel/1(in), Selector/1  "<v_Abs_Vehicle_CoG[x;y;z][km|h]>"
  BusCreator6/1 -> BusCreator1/1  "Linear"
  v_Vehicle_and_AngleSideSlip/1(v_Vehicle[km|h]) -> BusCreator4/2  "v_Total_Vehicle[km|h]"
  VectorLabel/1(out) -> BusCreator4/1
  Bus Selector/2 -> "[rad]_to_[deg]"/1  "<w_CoG_VehicleBody[x;y;z][rad|s]>"
  Bus Selector/3 -> BusCreator6/1  "<WheelBodyVelocity>"
  Bus Selector/4 -> BusCreator7/1  "<WheelBodyAngularVelocity>"
  Bus Selector/5 -> BusCreator7/2  "<WheelAngularVelocity>"
  Selector/1 -> v_Vehicle_and_AngleSideSlip/1(v_Vehicle[x;y][km|h])
  v_Vehicle_and_AngleSideSlip/2(Angle_SideSlip_Vehicle[deg]) -> BusCreator4/3  "Angle_SideSlip_Vehicle[deg]"

== system ASM_Traffic_new/DomainControl/DriverAssistance/Control/SoftECU_ACC/Soft_ECU_ACC/Map_Inputs/Maneuver/pos_edge_detection ==
  In1 : Inport
  Memory : Memory
  Relational Operator : RelationalOperator  Operator=>  OutDataTypeStr=boolean  InputSameDT=off
  Out1 : Outport  VectorParamsAs1DForOutWhenUnconnected=off
  wires:
  In1/1 -> Relational Operator/1, Memory/1
  Relational Operator/1 -> Out1/1
  Memory/1 -> Relational Operator/2

== system ASM_Traffic_new/DomainControl/DriverAssistance/Control/SoftECU_ACC/Soft_ECU_ACC/Map_Inputs/Maneuver/pos_edge_detection1 ==
  In1 : Inport
  Memory : Memory
  Relational Operator : RelationalOperator  Operator=>  OutDataTypeStr=boolean  InputSameDT=off
  Out1 : Outport  VectorParamsAs1DForOutWhenUnconnected=off
  wires:
  Memory/1 -> Relational Operator/2
  Relational Operator/1 -> Out1/1
  In1/1 -> Memory/1, Relational Operator/1

== system ASM_Traffic_new/DomainControl/DriverAssistance/Control/SoftECU_ACC/Soft_ECU_ACC/Map_Inputs/Maneuver/pos_edge_detection2 ==
  In1 : Inport
  Memory : Memory
  Relational Operator : RelationalOperator  Operator=>  OutDataTypeStr=boolean  InputSameDT=off
  Out1 : Outport  VectorParamsAs1DForOutWhenUnconnected=off
  wires:
  In1/1 -> Relational Operator/1, Memory/1
  Relational Operator/1 -> Out1/1
  Memory/1 -> Relational Operator/2

== system ASM_Traffic_new/DomainControl/DriverAssistance/Control/SoftECU_ACC/Soft_ECU_ACC/Map_Inputs/Maneuver/pos_edge_detection3 ==
  In1 : Inport
  Memory : Memory
  Relational Operator : RelationalOperator  Operator=>  OutDataTypeStr=boolean  InputSameDT=off
  Out1 : Outport  VectorParamsAs1DForOutWhenUnconnected=off
  wires:
  Memory/1 -> Relational Operator/2
  Relational Operator/1 -> Out1/1
  In1/1 -> Memory/1, Relational Operator/1

== system ASM_Traffic_new/Environment/GroundTruth/UserInterface/PAR_Plant/Fellow_Vehicles/Lightstates_Fellow1/Indicator_State[]/ASM_OSI_Mapping ==
  Fellow_TurnLights[] : Inport
  Table_ASM_To_OSI : Lookup_n-D  NumberOfTableDimensions=1  BreakpointsForDimension1=[0,1,2,3]  Table=[2,3,4,5]  InterpMethod=Nearest  InternalRulePriority=Speed  RndMeth=Simplest
  Indicator_State[] : Outport  VectorParamsAs1DForOutWhenUnconnected=off
  wires:
  Table_ASM_To_OSI/1 -> Indicator_State[]/1
  Fellow_TurnLights[]/1 -> Table_ASM_To_OSI/1

== system ASM_Traffic_new/Environment/GroundTruth/UserInterface/PAR_Plant/Fellow_Vehicles/Lightstates_Fellow10/Indicator_State[]/ASM_OSI_Mapping ==
  Fellow_TurnLights[] : Inport
  Table_ASM_To_OSI : Lookup_n-D  NumberOfTableDimensions=1  BreakpointsForDimension1=[0,1,2,3]  Table=[2,3,4,5]  InterpMethod=Nearest  InternalRulePriority=Speed  RndMeth=Simplest
  Indicator_State[] : Outport  VectorParamsAs1DForOutWhenUnconnected=off
  wires:
  Fellow_TurnLights[]/1 -> Table_ASM_To_OSI/1
  Table_ASM_To_OSI/1 -> Indicator_State[]/1

== system ASM_Traffic_new/Environment/GroundTruth/UserInterface/PAR_Plant/Fellow_Vehicles/Lightstates_Fellow11/Indicator_State[]/ASM_OSI_Mapping ==
  Fellow_TurnLights[] : Inport
  Table_ASM_To_OSI : Lookup_n-D  NumberOfTableDimensions=1  BreakpointsForDimension1=[0,1,2,3]  Table=[2,3,4,5]  InterpMethod=Nearest  InternalRulePriority=Speed  RndMeth=Simplest
  Indicator_State[] : Outport  VectorParamsAs1DForOutWhenUnconnected=off
  wires:
  Table_ASM_To_OSI/1 -> Indicator_State[]/1
  Fellow_TurnLights[]/1 -> Table_ASM_To_OSI/1

== system ASM_Traffic_new/Environment/GroundTruth/UserInterface/PAR_Plant/Fellow_Vehicles/Lightstates_Fellow12/Indicator_State[]/ASM_OSI_Mapping ==
  Fellow_TurnLights[] : Inport
  Table_ASM_To_OSI : Lookup_n-D  NumberOfTableDimensions=1  BreakpointsForDimension1=[0,1,2,3]  Table=[2,3,4,5]  InterpMethod=Nearest  InternalRulePriority=Speed  RndMeth=Simplest
  Indicator_State[] : Outport  VectorParamsAs1DForOutWhenUnconnected=off
  wires:
  Fellow_TurnLights[]/1 -> Table_ASM_To_OSI/1
  Table_ASM_To_OSI/1 -> Indicator_State[]/1

== system ASM_Traffic_new/Environment/GroundTruth/UserInterface/PAR_Plant/Fellow_Vehicles/Lightstates_Fellow13/Indicator_State[]/ASM_OSI_Mapping ==
  Fellow_TurnLights[] : Inport
  Table_ASM_To_OSI : Lookup_n-D  NumberOfTableDimensions=1  BreakpointsForDimension1=[0,1,2,3]  Table=[2,3,4,5]  InterpMethod=Nearest  InternalRulePriority=Speed  RndMeth=Simplest
  Indicator_State[] : Outport  VectorParamsAs1DForOutWhenUnconnected=off
  wires:
  Table_ASM_To_OSI/1 -> Indicator_State[]/1
  Fellow_TurnLights[]/1 -> Table_ASM_To_OSI/1

== system ASM_Traffic_new/Environment/GroundTruth/UserInterface/PAR_Plant/Fellow_Vehicles/Lightstates_Fellow14/Indicator_State[]/ASM_OSI_Mapping ==
  Fellow_TurnLights[] : Inport
  Table_ASM_To_OSI : Lookup_n-D  NumberOfTableDimensions=1  BreakpointsForDimension1=[0,1,2,3]  Table=[2,3,4,5]  InterpMethod=Nearest  InternalRulePriority=Speed  RndMeth=Simplest
  Indicator_State[] : Outport  VectorParamsAs1DForOutWhenUnconnected=off
  wires:
  Fellow_TurnLights[]/1 -> Table_ASM_To_OSI/1
  Table_ASM_To_OSI/1 -> Indicator_State[]/1

== system ASM_Traffic_new/Environment/GroundTruth/UserInterface/PAR_Plant/Fellow_Vehicles/Lightstates_Fellow15/Indicator_State[]/ASM_OSI_Mapping ==
  Fellow_TurnLights[] : Inport
  Table_ASM_To_OSI : Lookup_n-D  NumberOfTableDimensions=1  BreakpointsForDimension1=[0,1,2,3]  Table=[2,3,4,5]  InterpMethod=Nearest  InternalRulePriority=Speed  RndMeth=Simplest
  Indicator_State[] : Outport  VectorParamsAs1DForOutWhenUnconnected=off
  wires:
  Table_ASM_To_OSI/1 -> Indicator_State[]/1
  Fellow_TurnLights[]/1 -> Table_ASM_To_OSI/1

== system ASM_Traffic_new/Environment/GroundTruth/UserInterface/PAR_Plant/Fellow_Vehicles/Lightstates_Fellow16/Indicator_State[]/ASM_OSI_Mapping ==
  Fellow_TurnLights[] : Inport
  Table_ASM_To_OSI : Lookup_n-D  NumberOfTableDimensions=1  BreakpointsForDimension1=[0,1,2,3]  Table=[2,3,4,5]  InterpMethod=Nearest  InternalRulePriority=Speed  RndMeth=Simplest
  Indicator_State[] : Outport  VectorParamsAs1DForOutWhenUnconnected=off
  wires:
  Fellow_TurnLights[]/1 -> Table_ASM_To_OSI/1
  Table_ASM_To_OSI/1 -> Indicator_State[]/1

== system ASM_Traffic_new/Environment/GroundTruth/UserInterface/PAR_Plant/Fellow_Vehicles/Lightstates_Fellow17/Indicator_State[]/ASM_OSI_Mapping ==
  Fellow_TurnLights[] : Inport
  Table_ASM_To_OSI : Lookup_n-D  NumberOfTableDimensions=1  BreakpointsForDimension1=[0,1,2,3]  Table=[2,3,4,5]  InterpMethod=Nearest  InternalRulePriority=Speed  RndMeth=Simplest
  Indicator_State[] : Outport  VectorParamsAs1DForOutWhenUnconnected=off
  wires:
  Table_ASM_To_OSI/1 -> Indicator_State[]/1
  Fellow_TurnLights[]/1 -> Table_ASM_To_OSI/1

== system ASM_Traffic_new/Environment/GroundTruth/UserInterface/PAR_Plant/Fellow_Vehicles/Lightstates_Fellow18/Indicator_State[]/ASM_OSI_Mapping ==
  Fellow_TurnLights[] : Inport
  Table_ASM_To_OSI : Lookup_n-D  NumberOfTableDimensions=1  BreakpointsForDimension1=[0,1,2,3]  Table=[2,3,4,5]  InterpMethod=Nearest  InternalRulePriority=Speed  RndMeth=Simplest
  Indicator_State[] : Outport  VectorParamsAs1DForOutWhenUnconnected=off
  wires:
  Fellow_TurnLights[]/1 -> Table_ASM_To_OSI/1
  Table_ASM_To_OSI/1 -> Indicator_State[]/1

== system ASM_Traffic_new/Environment/GroundTruth/UserInterface/PAR_Plant/Fellow_Vehicles/Lightstates_Fellow19/Indicator_State[]/ASM_OSI_Mapping ==
  Fellow_TurnLights[] : Inport
  Table_ASM_To_OSI : Lookup_n-D  NumberOfTableDimensions=1  BreakpointsForDimension1=[0,1,2,3]  Table=[2,3,4,5]  InterpMethod=Nearest  InternalRulePriority=Speed  RndMeth=Simplest
  Indicator_State[] : Outport  VectorParamsAs1DForOutWhenUnconnected=off
  wires:
  Table_ASM_To_OSI/1 -> Indicator_State[]/1
  Fellow_TurnLights[]/1 -> Table_ASM_To_OSI/1

== system ASM_Traffic_new/Environment/GroundTruth/UserInterface/PAR_Plant/Fellow_Vehicles/Lightstates_Fellow2/Indicator_State[]/ASM_OSI_Mapping ==
  Fellow_TurnLights[] : Inport
  Table_ASM_To_OSI : Lookup_n-D  NumberOfTableDimensions=1  BreakpointsForDimension1=[0,1,2,3]  Table=[2,3,4,5]  InterpMethod=Nearest  InternalRulePriority=Speed  RndMeth=Simplest
  Indicator_State[] : Outport  VectorParamsAs1DForOutWhenUnconnected=off
  wires:
  Fellow_TurnLights[]/1 -> Table_ASM_To_OSI/1
  Table_ASM_To_OSI/1 -> Indicator_State[]/1

== system ASM_Traffic_new/Environment/GroundTruth/UserInterface/PAR_Plant/Fellow_Vehicles/Lightstates_Fellow20/Indicator_State[]/ASM_OSI_Mapping ==
  Fellow_TurnLights[] : Inport
  Table_ASM_To_OSI : Lookup_n-D  NumberOfTableDimensions=1  BreakpointsForDimension1=[0,1,2,3]  Table=[2,3,4,5]  InterpMethod=Nearest  InternalRulePriority=Speed  RndMeth=Simplest
  Indicator_State[] : Outport  VectorParamsAs1DForOutWhenUnconnected=off
  wires:
  Fellow_TurnLights[]/1 -> Table_ASM_To_OSI/1
  Table_ASM_To_OSI/1 -> Indicator_State[]/1

== system ASM_Traffic_new/Environment/GroundTruth/UserInterface/PAR_Plant/Fellow_Vehicles/Lightstates_Fellow21/Indicator_State[]/ASM_OSI_Mapping ==
  Fellow_TurnLights[] : Inport
  Table_ASM_To_OSI : Lookup_n-D  NumberOfTableDimensions=1  BreakpointsForDimension1=[0,1,2,3]  Table=[2,3,4,5]  InterpMethod=Nearest  InternalRulePriority=Speed  RndMeth=Simplest
  Indicator_State[] : Outport  VectorParamsAs1DForOutWhenUnconnected=off
  wires:
  Table_ASM_To_OSI/1 -> Indicator_State[]/1
  Fellow_TurnLights[]/1 -> Table_ASM_To_OSI/1

== system ASM_Traffic_new/Environment/GroundTruth/UserInterface/PAR_Plant/Fellow_Vehicles/Lightstates_Fellow22/Indicator_State[]/ASM_OSI_Mapping ==
  Fellow_TurnLights[] : Inport
  Table_ASM_To_OSI : Lookup_n-D  NumberOfTableDimensions=1  BreakpointsForDimension1=[0,1,2,3]  Table=[2,3,4,5]  InterpMethod=Nearest  InternalRulePriority=Speed  RndMeth=Simplest
  Indicator_State[] : Outport  VectorParamsAs1DForOutWhenUnconnected=off
  wires:
  Fellow_TurnLights[]/1 -> Table_ASM_To_OSI/1
  Table_ASM_To_OSI/1 -> Indicator_State[]/1

== system ASM_Traffic_new/Environment/GroundTruth/UserInterface/PAR_Plant/Fellow_Vehicles/Lightstates_Fellow23/Indicator_State[]/ASM_OSI_Mapping ==
  Fellow_TurnLights[] : Inport
  Table_ASM_To_OSI : Lookup_n-D  NumberOfTableDimensions=1  BreakpointsForDimension1=[0,1,2,3]  Table=[2,3,4,5]  InterpMethod=Nearest  InternalRulePriority=Speed  RndMeth=Simplest
  Indicator_State[] : Outport  VectorParamsAs1DForOutWhenUnconnected=off
  wires:
  Table_ASM_To_OSI/1 -> Indicator_State[]/1
  Fellow_TurnLights[]/1 -> Table_ASM_To_OSI/1

== system ASM_Traffic_new/Environment/GroundTruth/UserInterface/PAR_Plant/Fellow_Vehicles/Lightstates_Fellow24/Indicator_State[]/ASM_OSI_Mapping ==
  Fellow_TurnLights[] : Inport
  Table_ASM_To_OSI : Lookup_n-D  NumberOfTableDimensions=1  BreakpointsForDimension1=[0,1,2,3]  Table=[2,3,4,5]  InterpMethod=Nearest  InternalRulePriority=Speed  RndMeth=Simplest
  Indicator_State[] : Outport  VectorParamsAs1DForOutWhenUnconnected=off
  wires:
  Fellow_TurnLights[]/1 -> Table_ASM_To_OSI/1
  Table_ASM_To_OSI/1 -> Indicator_State[]/1
